simulink subsystem "Vehicle1D_Basic_refsub"  (R2026a)
settings: Solver=VariableStepAuto
undefined symbols (not defined in the file or in its folder): vehicle
libraries: nesl_utility x5, sdl_lib x1, fl_lib x1
settings Model: Creator=isaacito  LastModifiedBy=isaacito
settings SimscapeCC: SimscapeNominalValues="[{\"value\":\"1\",\"unit\":\"A\"},{\"value\":\"1\",\"unit\":\"bar\"},{\"value\":\"1\",\"unit\":\"cm^2\"},{\"value\":\"1\",\"unit\":\"cm^3/s\"},{\"value\":\"1\",\"unit\":\"kJ/kg\"},{\"value\":\"1\",\"unit\":\"kW\"},{\"value\":\"1\",\"unit\":\"l\"},{\"value\":\"1\",\"unit\":\"N\"},{\"value\":\"1\",\"unit\":\"N*m\"},{\"value\":\"1\",\"unit\":\"V\"}]"  SimscapeLogType=none  SimscapeLogDataHistory=5000.0

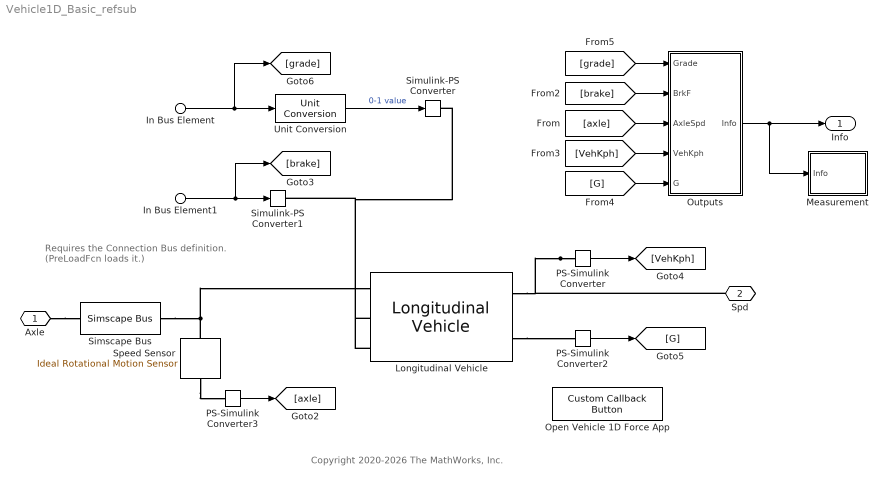
== system Vehicle1D_Basic_refsub ==
  note: Copyright 2020-2026 The MathWorks, Inc.
  note: Requires the Connection Bus definition.
      | (PreLoadFcn loads it.)
  In Bus Element : Inport  PortName=Inputs  Element=RoadGrade
      settings: AttributesFormatString=%<Unit>
  In Bus Element1 : Inport  PortName=Inputs  Element=BrakeForce
      settings: AttributesFormatString=%<Unit>
  Longitudinal Vehicle : sdl_lib/Tires & Vehicles/Longitudinal Vehicle  vehParamType=sdl.enum.VehicleParameterizationType.Regular  M_vehicle=vehicle.mass_kg kg  R_tireroll=vehicle.tireRollingRadius_m m  C_tireroll=vehicle.tireRollingCoeff  C_airdrag=vehicle.airDragCoeff  A_front=vehicle.frontalArea_m2 m^2  A_rl=vehicle.roadLoadA_N N  B_rl=vehicle.roadLoadB_N_per_kph N/(km/hr)  C_rl=vehicle.roadLoadC_N_per_kph2 N/(km/hr)^2  g=vehicle.gravAccel_m_per_s2 m/s^2  V_1=smoothing.vehicle_speedThreshold_kph km/hr  w_1=smoothing.vehicle_axleSpeedThreshold_rpm rpm  ShowBrakeIn=simscape.enum.onoff.on  ShowSlopeIn=simscape.enum.onoff.on  SlopeInputType=sdl.enum.VehicleLongitudinalRoadSlopeInputType.Grade  ShowWindIn=simscape.enum.onoff.off  ShowGOut=simscape.enum.onoff.on  air_density=1.184 kg/m^3  V_x_specify=on  V_x_priority=High  V_x=initial.vehicle_speed_kph km/hr  V_x_nominal_specify=off  V_x_nominal_value=1  V_x_nominal_unit=m/s  trq_specify=off  trq_priority=None  trq=0 N*m  trq_nominal_specify=off  trq_nominal_value=1  trq_nominal_unit=N*m  w_specify=off  w_priority=None  w=0 rad/s  w_nominal_specify=off  w_nominal_value=1  w_nominal_unit=rad/s
      settings: AttributesFormatString=|
      | %<V_x> [%<V_x_unit>]
      | Priority: %<V_x_priority>
  Measurement : Subsystem
  Open Vehicle 1D Force App : CustomCallbackButton  Configuration="{\"components\":[{\"name\":\"BackgroundImageComponent\",\"settings\":{\"image\":{\"size\":[0,0],\"src\":\"default\",\"srcOrientation\":\"Right\"},\"position\":[0,0,1,1]}},{\"name\":\"ButtonStateComponent\",\"settings\":{\"buttonType\":\"momentary\",\"clickFcn\":\"disp(\\\"Opening app\\\")\\nbevutil1_Vehicle1DForceApp(BlockPath=(gcs + \\\"\\/Longitudinal Vehicle\\\"))\",\"onValue\":1,\"position\":[0,0,1,1],\"pressDelay\":\"500\",\"pressFcn\":\"\",\"repeatInterval\":\"0\",\"states\":[{\"horizontalAlignment\":\"center\",\"image\":{\"position\":[0,0,1,1],\"size\":[1,1],\"src\":\"default\",\"srcOrientation\":\"Right\"},\"label\":{\"color\":[0.01176470588,0.01176470588,0.01176470588,1],\"icon\":{\"size\":[0,0],\"src\":\"default\",\"srcOrientation\":\"Right\"},\"iconOffset\":0,\"iconPlacement\":\"left\",\"opacity\":1,\"show\":true,\"text\":{\"content\":\"Open App\",\"font\":\"Helvetica\"}},\"labelOffset\":[0,0],\"verticalAlignment\":\"middle\"},{\"horizontalAlignment\":\"center\",\"image\":{\"position\":[0,0,1,1],\"size\":[1,1],\"src\":\"default\",\"srcOrientation\":\"Right\"},\"label\":{\"color\":[0.01176470588,0.01176470588,0.01176470588,1],\"icon\":{\"size\":[0,0],\"src\":\"default\",\"srcOrientation\":\"Right\"},\"iconOffset\":0,\"iconPlacement\":\"left\",\"opacity\":1,\"show\":true,\"text\":{\"content\":\"Open App\",\"font\":\"Helvetica\"}},\"labelOffset\":[0,0],\"verticalAlignment\":\"middle\"},{\"horizontalAlignment\":\"center\",\"image\":{\"position\":[0,0,1,1],\"size\":[1,1],\"src\":\"default\",\"srcOrientation\":\"Right\"},\"label\":{\"color\":[0.01176470588,0.01176470588,0.01176470588,1],\"icon\":{\"size\":[0,0],\"src\":\"default\",\"srcOrientation\":\"Right\"},\"iconOffset\":0,\"iconPlacement\":\"left\",\"opacity\":1,\"show\":true,\"text\":{\"content\":\"Open App\",\"font\":\"Helvetica\"}},\"labelOffset\":[0,0],\"verticalAlignment\":\"middle\"},{\"horizontalAlignment\":\"center\",\"image\":{\"position\":[0,0,1,1],\"size\":[1,1],\"src\":\"default\",\"srcOrientation\":\"Right\"},\"label\":{\"color\":[0.01176470588,0.01176470588,0.01176470588,1],\"icon\":{\"size\":[0,0],\"src\":\"default\",\"srcOrientation\":\"Right\"},\"iconOffset\":0,\"iconPlacement\":\"left\",\"opacity\":1,\"show\":true,\"text\":{\"content\":\"Open App\",\"font\":\"Helvetica\"}},\"labelOffset\":[0,0],\"verticalAlignment\":\"middle\"}]}},{\"name\":\"ForegroundImageComponent\",\"settings\":{\"image\":{\"size\":[0,0],\"src\":\"default\",\"srcOrientation\":\"Right\"},\"isForeground\":1,\"position\":[0,0,1,1]}}],\"derived\":{\"blockParameters\":{\"AutoActivate\":true,\"ButtonText\":\"Open App\",\"ButtonType\":\"Momentary\",\"ClickFcn\":\"disp(\\\"Opening app\\\")\\nbevutil1_Vehicle1DForceApp(BlockPath=(gcs + \\\"\\/Longitudinal Vehicle\\\"))\",\"OnValue\":1,\"PressDelay\":\"500\",\"PressFcn\":\"\",\"RepeatInterval\":\"0\",\"fixedAspectRatio\":\"off\"}},\"settings\":{\"BindingType\":\"standalone\",\"autoActivate\":true,\"backgroundColor\":[244,244,244,1],\"backgroundOffset\":0.2,\"backgroundOpacity\":1,\"fixedAspectRatio\":\"off\",\"foregroundColor\":[0.01176470588,0.01176470588,0.01176470588,1],\"migratedFromLegacy\":true,\"useBackgroundColor\":true,\"variant\":\"callback\",\"version\":\"R2025a\"},\"type\":\"Button\"}"  CustomBackgroundColor="{\"color\":[0.9568627451,0.9568627451,0.9568627451],\"show\":true}"
  Outputs : Subsystem
  PS-Simulink Converter : nesl_utility/PS-Simulink Converter  PhysicalDomain=network_engine_domain  SubClassName=ps_output  LeftPortType=input  RightPortType=output  PseudoPeriodic=off  Frequencies=[]  VectorFormat=1-D array  Unit=km/hr  AffineConversion=off
  PS-Simulink Converter2 : nesl_utility/PS-Simulink Converter  PhysicalDomain=network_engine_domain  SubClassName=ps_output  LeftPortType=input  RightPortType=output  PseudoPeriodic=off  Frequencies=[]  VectorFormat=1-D array  Unit=1  AffineConversion=off
  PS-Simulink Converter3 : nesl_utility/PS-Simulink Converter  PhysicalDomain=network_engine_domain  SubClassName=ps_output  LeftPortType=input  RightPortType=output  PseudoPeriodic=off  Frequencies=[]  VectorFormat=1-D array  Unit=rpm  AffineConversion=off
  Simscape Bus : SimscapeBus  HierarchyStrings=AngSpd  ConnectionType=Bus: Bus_Rotational
      settings: AttributesFormatString=%<ConnectionType>
  Simulink-PS Converter : nesl_utility/Simulink-PS Converter  PhysicalDomain=network_engine_domain  SubClassName=ps_input  LeftPortType=input  RightPortType=output  PseudoPeriodic=off  Frequencies=[]  NoiseDistribution=none  NoiseParameters=[]  Unit=1  AffineConversion=off  FilteringAndDerivatives=filter  SimscapeFilterOrder=1  InputFilterTimeConstant=0.001  UdotUserProvided=0
  Simulink-PS Converter1 : nesl_utility/Simulink-PS Converter  PhysicalDomain=network_engine_domain  SubClassName=ps_input  LeftPortType=input  RightPortType=output  PseudoPeriodic=off  Frequencies=[]  NoiseDistribution=none  NoiseParameters=[]  Unit=N  AffineConversion=off  FilteringAndDerivatives=filter  SimscapeFilterOrder=1  InputFilterTimeConstant=0.001  UdotUserProvided=0
  Speed Sensor : fl_lib/Mechanical/Mechanical Sensors/Ideal Rotational Motion Sensor  reference=foundation.enum.MeasurementReference.absolute  acceleration_port=false  velocity_port=true  position_port=false  wrap_angle=simscape.enum.onoff.off  offset=0 rad
  Unit Conversion : UnitConversion  OutputType=Inherit: Inherit via back propagation
  Axle : PMIOPort  Side=Left
  Spd : PMIOPort  Port=2  Side=Right
  Info : Outport
  wires:
  PS-Simulink Converter3/1 -> [axle]
  Unit Conversion/1 -> Simulink-PS Converter/1  "0-1 value"
  In Bus Element1/1 -> Simulink-PS Converter1/1, [brake]
  In Bus Element/1 -> Unit Conversion/1, [grade]
  PS-Simulink Converter2/1 -> [G]
  PS-Simulink Converter/1 -> [VehKph]
  Outputs/1(Info) -> Measurement/1(Info), Info/1
  [G] -> Outputs/5(G)
  [grade] -> Outputs/1(Grade)
  [VehKph] -> Outputs/4(VehKph)
  [axle] -> Outputs/3(AxleSpd)
  [brake] -> Outputs/2(BrkF)
  connections:
  Speed Sensor/LConn1 -- Simscape Bus/LConn1 -- Longitudinal Vehicle/LConn1
  PS-Simulink Converter/LConn1 -- Spd/RConn1 -- Longitudinal Vehicle/RConn1
  Speed Sensor/RConn1 -- PS-Simulink Converter3/LConn1
  Longitudinal Vehicle/LConn2 -- Simulink-PS Converter1/RConn1
  Longitudinal Vehicle/LConn3 -- Simulink-PS Converter/RConn1
  Longitudinal Vehicle/RConn2 -- PS-Simulink Converter2/LConn1
  Axle/RConn1 -- Simscape Bus/RConn1

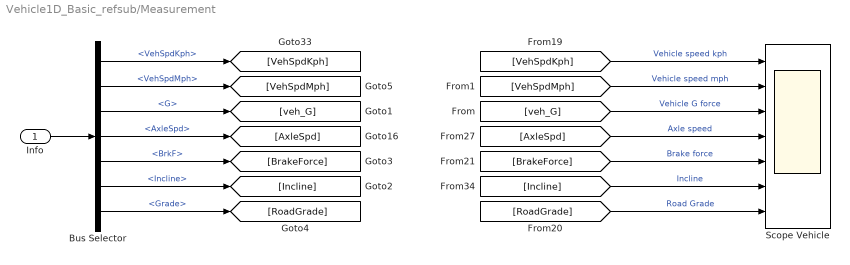
== system Vehicle1D_Basic_refsub/Measurement ==
  Info : Inport
  Bus Selector : BusSelector  OutputSignals=VehSpdKph,VehSpdMph,G,AxleSpd,BrkF,Incline,Grade
  Scope Vehicle : Scope  NumInputPorts=7
      settings: ActiveDisplayYMinimum=-12.00926  ActiveDisplayYMaximum=102.7511
  wires:
  Bus Selector/6 -> [Incline]  "<Incline>"
  Bus Selector/7 -> [RoadGrade]  "<Grade>"
  Bus Selector/5 -> [BrakeForce]  "<BrkF>"
  Bus Selector/4 -> [AxleSpd]  "<AxleSpd>"
  Bus Selector/3 -> [veh_G]  "<G>"
  Bus Selector/2 -> [VehSpdMph]  "<VehSpdMph>"
  Bus Selector/1 -> [VehSpdKph]  "<VehSpdKph>"
  Info/1 -> Bus Selector/1
  [VehSpdMph] -> Scope Vehicle/2  "Vehicle speed mph"
  [RoadGrade] -> Scope Vehicle/7  "Road Grade"
  [Incline] -> Scope Vehicle/6  "Incline"
  [BrakeForce] -> Scope Vehicle/5  "Brake force"
  [AxleSpd] -> Scope Vehicle/4  "Axle speed"
  [veh_G] -> Scope Vehicle/3  "Vehicle G force"
  [VehSpdKph] -> Scope Vehicle/1  "Vehicle speed kph"

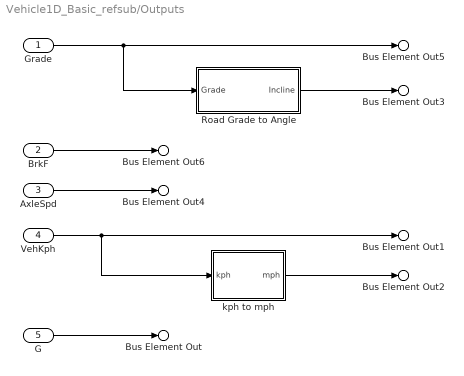
== system Vehicle1D_Basic_refsub/Outputs ==
  Grade : Inport  Unit=%
      settings: AttributesFormatString=%<Unit>
  BrkF : Inport  Port=2  Unit=N
      settings: AttributesFormatString=%<Unit>
  AxleSpd : Inport  Port=3  Unit=rpm
      settings: AttributesFormatString=%<Unit>
  VehKph : Inport  Port=4  Unit=km/hr
      settings: AttributesFormatString=%<Unit>
  G : Inport  Port=5  Unit=1
      settings: AttributesFormatString=%<Unit>
  Road Grade to Angle : Subsystem
  kph to mph : Subsystem
  Bus Element Out : Outport  PortName=Info  Element=G
      settings: AttributesFormatString=%<Unit>
  Bus Element Out1 : Outport  PortName=Info  Element=VehSpdKph
      settings: AttributesFormatString=%<Unit>
  Bus Element Out2 : Outport  PortName=Info  Element=VehSpdMph
      settings: AttributesFormatString=%<Unit>
  Bus Element Out3 : Outport  PortName=Info  Element=Incline
      settings: AttributesFormatString=%<Unit>
  Bus Element Out4 : Outport  PortName=Info  Element=AxleSpd
      settings: AttributesFormatString=%<Unit>
  Bus Element Out5 : Outport  PortName=Info  Element=Grade
      settings: AttributesFormatString=%<Unit>
  Bus Element Out6 : Outport  PortName=Info  Element=BrkF
      settings: AttributesFormatString=%<Unit>
  wires:
  kph to mph/1(mph) -> Bus Element Out2/1
  Road Grade to Angle/1(Incline) -> Bus Element Out3/1
  Grade/1 -> Bus Element Out5/1, Road Grade to Angle/1(Grade)
  BrkF/1 -> Bus Element Out6/1
  G/1 -> Bus Element Out/1
  VehKph/1 -> Bus Element Out1/1, kph to mph/1(kph)
  AxleSpd/1 -> Bus Element Out4/1

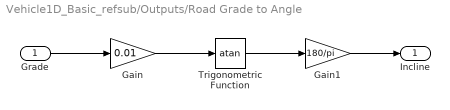
== system Vehicle1D_Basic_refsub/Outputs/Road Grade to Angle ==
  Grade : Inport  Unit=%
      settings: AttributesFormatString=%<Unit>
  Gain : Gain  Gain=0.01
  Gain1 : Gain  Gain=180/pi
  Trigonometric Function : Trigonometry  Operator=atan
  Incline : Outport  Unit=deg
      settings: AttributesFormatString=%<Unit>
  wires:
  Gain/1 -> Trigonometric Function/1
  Grade/1 -> Gain/1
  Trigonometric Function/1 -> Gain1/1
  Gain1/1 -> Incline/1

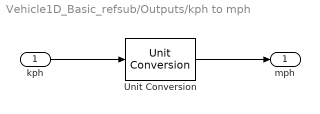
== system Vehicle1D_Basic_refsub/Outputs/kph to mph ==
  kph : Inport  Unit=km/h
  Unit Conversion : UnitConversion
  mph : Outport  Unit=mph
  wires:
  Unit Conversion/1 -> mph/1
  kph/1 -> Unit Conversion/1
